simulink library "tip_assist_lib_support"  (Simulink 9.0)
settings: Solver=VariableStepAuto  StartTime=0.0  StopTime=10.0  RelTol=1e-3
undefined symbols (not defined in the file): g, timestep, TipAssistAdvEcmError_t, TipAssistCpmTipOffMode_t, TipAssistLiveWeighStatus_t, TipAssistPayloadType_t, TipAssistSecPfwStatus_t, TipAssistUnsecPfwStatus_t, toa_appNumber, toa_expectedBucketAngNoise, toa_imu_lpf_cutoff_hz, toa_imuBasicOrient, toa_liftBoreDia, toa_liftRodDia, toa_liveLpfCutoffHz, toa_liveSpillRateLpfCutoffHz, toa_mcGroundCombBucketAng, toa_mcGroundCombLiftNormAng, toa_mcGroundLiftNormAng, toa_noSlidingAngle, toa_payload_target_ov_val, toa_payloadTargetMin, toa_pfwLpfCutoffHz, toa_pfwResetLpfCutoffHz, toa_pfwResetStatsBound, toa_pfwResetStatsConf, toa_pfwTiltNormRackThresh, toa_pfwTravelExtentLower, toa_pfwTravelExtentUpper, toa_ratedPayload, toa_reposeMarginAng, toa_sendCpmLiveLpfCutoffHz, toa_sendToCpmMinPrecision, toa_tiltBoreDia, toa_tiltNumCyl, toa_tiltRodDia, toa_toolBcAngle, toa_toolBcLength
libraries: lib_CATutils_Utilities_ApplyName_v2 x113, simulink x18, tip_assist_lib x14, lib_CATutils_Filters_1Pole_LowPass x6, simulink_extras x5, lib_CATutils_Override x3, lib_CATutils_Hysteresis_Latch x3, lib_CATutils_Timer_Countdown x3, tip_assist_lib_support x2
(part 1 of 4)
settings Model: Creator=CurriSD  LastModifiedBy=CurriSD

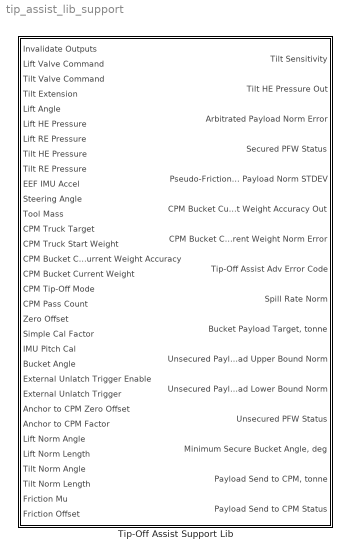
== system tip_assist_lib_support ==
  Tip-Off Assist Support Lib : Subsystem

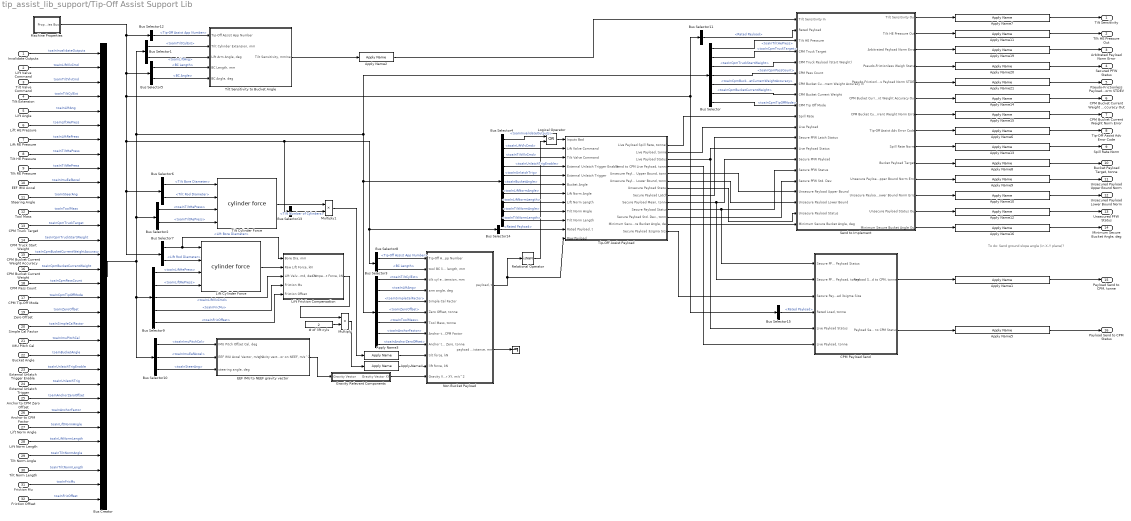
== system tip_assist_lib_support/Tip-Off Assist Support Lib ==
  note: To do: Send ground slope angle (in X-Y plane)?
  Invalidate Outputs : Inport
  Lift Valve Command : Inport  Port=2
  Tilt Valve Command : Inport  Port=3
  Tilt Extension : Inport  Port=4
  Lift Angle : Inport  Port=5
  Lift HE Pressure : Inport  Port=6
  Lift RE Pressure : Inport  Port=7
  Tilt HE Pressure : Inport  Port=8
  Tilt RE Pressure : Inport  Port=9
  EEF IMU Accel : Inport  Port=10
  Steering Angle : Inport  Port=11
  Tool Mass : Inport  Port=12
  CPM Truck Target : Inport  Port=13
  CPM Truck Start Weight : Inport  Port=14
  CPM Bucket Current Weight Accuracy : Inport  Port=15
  CPM Bucket Current Weight : Inport  Port=16
  CPM Tip-Off Mode : Inport  Port=17
  CPM Pass Count : Inport  Port=18
  Zero Offset : Inport  Port=19
  Simple Cal Factor : Inport  Port=20
  IMU Pitch Cal : Inport  Port=21
  Bucket Angle : Inport  Port=22
  External Unlatch Trigger Enable : Inport  Port=23
  External Unlatch Trigger : Inport  Port=24
  Anchor to CPM Zero Offset : Inport  Port=25
  Anchor to CPM Factor : Inport  Port=26
  Lift Norm Angle : Inport  Port=27
  Lift Norm Length : Inport  Port=28
  Tilt Norm Angle : Inport  Port=29
  Tilt Norm Length : Inport  Port=30
  Friction Mu : Inport  Port=31
  Friction Offset : Inport  Port=32
  " " : Terminator
  # of lift cyls : Constant  Value=2  OutDataTypeStr=single
  Apply Name1 : lib_CATutils_Utilities_ApplyName_v2/Apply Name  sigLabel='toa_outSendCpmPayload'  enTst=true
  Apply Name10 : lib_CATutils_Utilities_ApplyName_v2/Apply Name  sigLabel='toa_outUnsecPayloadNormLow'  enTst=true
  Apply Name11 : lib_CATutils_Utilities_ApplyName_v2/Apply Name  sigLabel='toa_outTiltHePress'  enTst=true
  Apply Name12 : lib_CATutils_Utilities_ApplyName_v2/Apply Name  sigLabel='toa_outUnsecPayloadStatus'  enTst=true
  Apply Name13 : lib_CATutils_Utilities_ApplyName_v2/Apply Name  sigLabel='toa_outSpillRateNorm'  enTst=true
  Apply Name14 : lib_CATutils_Utilities_ApplyName_v2/Apply Name  sigLabel='toa_outCpmAccu'  enTst=true
  Apply Name15 : lib_CATutils_Utilities_ApplyName_v2/Apply Name  sigLabel='toa_outCpmPayloadNormError'  enTst=true
  Apply Name16 : lib_CATutils_Utilities_ApplyName_v2/Apply Name  sigLabel='toa_outMinSecBucketAng'  enTst=true
  Apply Name19 : lib_CATutils_Utilities_ApplyName_v2/Apply Name  sigLabel='toa_outPayloadArbNormError'  enTst=true
  Apply Name2 : lib_CATutils_Utilities_ApplyName_v2/Apply Name  sigLabel='toa_tiltSensitivity'  enTst=true
  Apply Name20 : lib_CATutils_Utilities_ApplyName_v2/Apply Name  sigLabel='toa_outPfwStat'  enTst=true
  Apply Name21 : lib_CATutils_Utilities_ApplyName_v2/Apply Name  sigLabel='toa_outPfwPayloadNormStdev'  enTst=true
  Apply Name3 : lib_CATutils_Utilities_ApplyName_v2/Apply Name  sigLabel='toa_tiltForce'  enTst=true
  Apply Name4 : lib_CATutils_Utilities_ApplyName_v2/Apply Name  sigLabel='toa_liftForce'  enTst=true
  Apply Name5 : lib_CATutils_Utilities_ApplyName_v2/Apply Name  sigLabel='toa_outSendCpmStatus'  enTst=true
  Apply Name6 : lib_CATutils_Utilities_ApplyName_v2/Apply Name  sigLabel='toa_outAdvErrorCode'  enTst=true
  Apply Name7 : lib_CATutils_Utilities_ApplyName_v2/Apply Name  sigLabel='toa_outTiltSensToBucket'  enTst=true
  Apply Name8 : lib_CATutils_Utilities_ApplyName_v2/Apply Name  sigLabel='toa_outBucketPayloadTarget'  enTst=true
  Apply Name9 : lib_CATutils_Utilities_ApplyName_v2/Apply Name  sigLabel='toa_outUnsecPayloadNormUp'  enTst=true
  Bus Creator : BusCreator  Inputs=32
  Bus Selector : BusSelector  OutputSignals=toaInTiltHePress,toaInCpmTruckTarget,taoInCpmTruckStartWeight,toaInCpmPassCount,toaInCpmBucketCurrentWeightAccuracy,toaInCpmBucketCurrentWeight,toaInCpmTipOffMode
  Bus Selector1 : BusSelector  OutputSignals=toaInTiltCylExt,toaInLiftAng
  Bus Selector10 : BusSelector  OutputSignals=toaInImuPitchCal,toaInImuEefAccel,toaInSteerAng
  Bus Selector11 : BusSelector  OutputSignals=Rated Payload
  Bus Selector12 : BusSelector  OutputSignals=Tip-Off Assist App Number
  Bus Selector13 : BusSelector  OutputSignals=Tilt Number of Cylinders
  Bus Selector14 : BusSelector  OutputSignals=Rated Payload
  Bus Selector15 : BusSelector  OutputSignals=Rated Payload
  Bus Selector2 : BusSelector  OutputSignals=toaInTiltHePress,toaInTiltRePress
  Bus Selector3 : BusSelector  OutputSignals=toaInTiltCylExt,toaInLiftAng,toaInSimpleCalFactor,toaInZeroOffset,toaInToolMass,toaInAnchorFactor,toaInAnchorZeroOffset
  Bus Selector4 : BusSelector  OutputSignals=toaInInvalidateOutputs,toaInLiftVlvCmd,toaInTiltVlvCmd,toaInUnlatchTrigEnable,toaInUnlatchTrig,toaInBucketAngle,toaInLiftNormAngle,toaInLiftNormLength,toaInTiltNormAngle,toaInTiltNormLength
  Bus Selector5 : BusSelector  OutputSignals=BC Length,BC Angle
  Bus Selector6 : BusSelector  OutputSignals=Tilt Bore Diameter,Tilt Rod Diameter
  Bus Selector8 : BusSelector  OutputSignals=Tip-Off Assist App Number,BC Length
  Bus Selector9 : BusSelector  OutputSignals=toaInLiftHePress,toaInLiftRePress,toaInLiftVlvCmd,toaInFricMu,toaInFricOffset
  Bus Selector7 : BusSelector  OutputSignals=Lift Bore Diameter,Lift Rod Diameter
  CPM Payload Send : Subsystem
  EEF IMU to NEEF gravity vector : Subsystem
  Gravity Relevant Components : Subsystem
  Lift Cylinder Force : tip_assist_lib/cylinder force
  Lift Friction Compensation : Subsystem
  Logical Operator : Logic  Operator=OR  AllPortsSameDT=off  OutDataTypeStr=boolean
  Machine Properties : Subsystem
  Multiply : Product  SaturateOnIntegerOverflow=on  RndMeth=Zero  InputSameDT=on  OutDataTypeStr=Inherit: Same as first input
  Multiply1 : Product  SaturateOnIntegerOverflow=on  RndMeth=Zero  InputSameDT=on  OutDataTypeStr=Inherit: Same as first input
  Non Bucket Payload : Subsystem
  Relational Operator : RelationalOperator  Operator=isNaN  OutDataTypeStr=boolean  RndMeth=Simplest
  Send to Implement : Subsystem
  Tilt Cylinder Force : tip_assist_lib/cylinder force
  Tilt Sensitivity to Bucket Angle : Subsystem
  Tip-Off Assist Payload : Subsystem
  Tilt Sensitivity : Outport
  Tilt HE Pressure Out : Outport  Port=2
  Arbitrated Payload Norm Error : Outport  Port=3
  Secured PFW Status : Outport  Port=4
  Pseudo-Frictionless Payload Norm STDEV : Outport  Port=5
  CPM Bucket Current Weight Accuracy Out : Outport  Port=6
  CPM Bucket Current Weight Norm Error : Outport  Port=7
  Tip-Off Assist Adv Error Code : Outport  Port=8
  Spill Rate Norm : Outport  Port=9
  "Bucket Payload Target, tonne" : Outport  Port=10
  Unsecured Payload Upper Bound Norm : Outport  Port=11
  Unsecured Payload Lower Bound Norm : Outport  Port=12
  Unsecured PFW Status : Outport  Port=13
  "Minimum Secure Bucket Angle, deg" : Outport  Port=14
  "Payload Send to CPM, tonne" : Outport  Port=15
  Payload Send to CPM Status : Outport  Port=16
  wires:
  Apply Name4/1 -> Non Bucket Payload/11("lift force, kN")
  Apply Name3/1 -> Non Bucket Payload/10("tilt force, kN")
  Apply Name2/1 -> Send to Implement/1(Tilt Sensitivity In)
  Non Bucket Payload/2("payload distance, mm") -> " "/1
  Non Bucket Payload/1("payload, t") -> Relational Operator/1, Tip-Off Assist Payload/12(Raw Payload)
  Send to Implement/2(Tilt HE Pressure Out) -> Apply Name11/1
  Bus Selector/1 -> Send to Implement/3(Tilt HE Pressure)  "<toaInTiltHePress>"
  Bus Selector/6 -> Send to Implement/8(CPM Bucket Current Weight)  "<toaInCpmBucketCurrentWeight>"
  Bus Selector/5 -> Send to Implement/7(CPM Bucket Current Weight Accuracy In)  "<toaInCpmBucketCurrentWeightAccuracy>"
  Bus Selector/3 -> Send to Implement/5(CPM Truck Payload (Start Weight))  "<taoInCpmTruckStartWeight>"
  Bus Selector/7 -> Send to Implement/9(CPM Tip Off Mode)  "<toaInCpmTipOffMode>"
  Bus Selector/2 -> Send to Implement/4(CPM Truck Target)  "<toaInCpmTruckTarget>"
  Bus Selector3/5 -> Non Bucket Payload/7("Tool Mass, tonne")  "<toaInToolMass>"
  Tool Mass/1 -> Bus Creator/12  "toaInToolMass"
  Bus Selector10/3 -> EEF IMU to NEEF gravity vector/3("steering angle, deg")  "<toaInSteerAng>"
  Bus Selector10/2 -> EEF IMU to NEEF gravity vector/2("EEF IMU Accel Vector, m/s^2")  "<toaInImuEefAccel>"
  Bus Selector9/2 -> Lift Cylinder Force/4  "<toaInLiftRePress>"
  Bus Selector9/1 -> Lift Cylinder Force/3  "<toaInLiftHePress>"
  Bus Selector2/2 -> Tilt Cylinder Force/4  "<toaInTiltRePress>"
  Bus Selector2/1 -> Tilt Cylinder Force/3  "<toaInTiltHePress>"
  Lift Angle/1 -> Bus Creator/5  "toaInLiftAng"
  Tilt Extension/1 -> Bus Creator/4  "toaInTiltCylExt"
  Tilt Valve Command/1 -> Bus Creator/3  "toaInTiltVlvCmd"
  Lift Valve Command/1 -> Bus Creator/2  "toaInLiftVlvCmd"
  Lift RE Pressure/1 -> Bus Creator/7  "toaInLiftRePress"
  Bus Selector7/2 -> Lift Cylinder Force/2  "<Lift Rod Diameter>"
  Bus Selector4/3 -> Tip-Off Assist Payload/3(Tilt Valve Command)  "<toaInTiltVlvCmd>"
  Bus Selector4/2 -> Tip-Off Assist Payload/2(Lift Valve Command)  "<toaInLiftVlvCmd>"
  Tip-Off Assist Payload/1("Live Payload Spill Rate, tonne/s") -> Send to Implement/10(Spill Rate)
  Tip-Off Assist Payload/2("Live Payload, tonne") -> Send to Implement/11(Live Payload)
  Tip-Off Assist Payload/10(Secure Payload Status) -> CPM Payload Send/1(Secure PFW Payload Status), Send to Implement/15(Secure PFW Status)
  Bus Creator/1 -> Bus Selector1/1, Bus Selector3/1, Bus Selector4/1, Bus Selector/1, Bus Selector2/1, Bus Selector9/1, Bus Selector10/1
  Send to Implement/9(Spill Rate Norm) -> Apply Name13/1
  Send to Implement/8(Tip-Off Assist Adv Error Code) -> Apply Name6/1
  Send to Implement/4(Pseudo-Frictionless Weigh Status) -> Apply Name20/1
  Send to Implement/7(CPM Bucket Current Weight Norm Error) -> Apply Name15/1
  Send to Implement/6(CPM Bucket Current Weight Accuracy Out) -> Apply Name14/1
  Bus Selector8/2 -> Non Bucket Payload/2("tool BC link length, mm")  "<BC Length>"
  Bus Selector7/1 -> Lift Cylinder Force/1, Lift Friction Compensation/1("Bore Dia, mm")  "<Lift Bore Diameter>"
  Bus Selector6/2 -> Tilt Cylinder Force/2  "<Tilt Rod Diameter>"
  Bus Selector6/1 -> Tilt Cylinder Force/1  "<Tilt Bore Diameter>"
  Machine Properties/1(Properties Bus) -> Bus Selector12/1, Bus Selector11/1, Bus Selector15/1, Bus Selector7/1, Bus Selector6/1, Bus Selector8/1, Bus Selector14/1, Bus Selector13/1, Bus Selector5/1
  Bus Selector5/1 -> Tilt Sensitivity to Bucket Angle/4("BC Length, mm")  "<BC Length>"
  Bus Selector5/2 -> Tilt Sensitivity to Bucket Angle/5("BC Angle, deg")  "<BC Angle>"
  Gravity Relevant Components/1(Gravity Vector XY) -> Non Bucket Payload/12("Gravity Vector XY, m/s^2")
  EEF IMU to NEEF gravity vector/1("gravity vector on NEEF, m/s^2") -> Gravity Relevant Components/1(Gravity Vector)
  Bus Selector3/2 -> Non Bucket Payload/4("arm angle, deg")  "<toaInLiftAng>"
  Bus Selector3/1 -> Non Bucket Payload/3("tilt cyl extension, mm")  "<toaInTiltCylExt>"
  Bus Selector1/2 -> Tilt Sensitivity to Bucket Angle/3("Lift Arm Angle, deg")  "<toaInLiftAng>"
  Bus Selector1/1 -> Tilt Sensitivity to Bucket Angle/2("Tilt Cylinder Extension, mm")  "<toaInTiltCylExt>"
  Send to Implement/1(Tilt Sensitivity Out) -> Apply Name7/1
  Send to Implement/5(Pseudo-Frictionless Payload Norm STDEV) -> Apply Name21/1
  Send to Implement/3(Arbitrated Payload Norm Error) -> Apply Name19/1
  Tilt Sensitivity to Bucket Angle/1("Tilt Sensitivity, mm/rad") -> Apply Name2/1
  Steering Angle/1 -> Bus Creator/11  "toaInSteerAng"
  EEF IMU Accel/1 -> Bus Creator/10  "toaInImuEefAccel"
  # of lift cyls/1 -> Multiply/2
  Tilt Cylinder Force/1 -> Multiply1/1
  Multiply/1 -> Apply Name4/1
  Tilt RE Pressure/1 -> Bus Creator/9  "toaInTiltRePress"
  Lift HE Pressure/1 -> Bus Creator/6  "toaInLiftHePress"
  Tilt HE Pressure/1 -> Bus Creator/8  "toaInTiltHePress"
  Apply Name7/1 -> Tilt Sensitivity/1
  Apply Name11/1 -> Tilt HE Pressure Out/1
  Apply Name19/1 -> Arbitrated Payload Norm Error/1
  Apply Name20/1 -> Secured PFW Status/1
  Apply Name21/1 -> Pseudo-Frictionless Payload Norm STDEV/1
  Apply Name14/1 -> CPM Bucket Current Weight Accuracy Out/1
  Apply Name15/1 -> CPM Bucket Current Weight Norm Error/1
  Apply Name6/1 -> Tip-Off Assist Adv Error Code/1
  Apply Name13/1 -> Spill Rate Norm/1
  Bus Selector13/1 -> Multiply1/2  "<Tilt Number of Cylinders>"
  Multiply1/1 -> Apply Name3/1
  CPM Payload Send/1("Payload Send to CPM, tonne") -> Apply Name1/1
  CPM Payload Send/2(Payload Send to CPM Status) -> Apply Name5/1
  Invalidate Outputs/1 -> Bus Creator/1  "toaInInvalidateOutputs"
  CPM Truck Target/1 -> Bus Creator/13  "toaInCpmTruckTarget"
  CPM Truck Start Weight/1 -> Bus Creator/14  "taoInCpmTruckStartWeight"
  CPM Bucket Current Weight Accuracy/1 -> Bus Creator/15  "toaInCpmBucketCurrentWeightAccuracy"
  CPM Bucket Current Weight/1 -> Bus Creator/16  "toaInCpmBucketCurrentWeight"
  Bus Selector4/1 -> Logical Operator/1  "<toaInInvalidateOutputs>"
  Tip-Off Assist Payload/3(Live Payload Status) -> Send to Implement/13(Live Payload Status), CPM Payload Send/5(Live Payload Status)
  Bus Selector11/1 -> Send to Implement/2(Rated Payload)  "<Rated Payload>"
  Bus Selector8/1 -> Non Bucket Payload/1(Tip-Off Assist App Number)  "<Tip-Off Assist App Number>"
  Bus Selector12/1 -> Tilt Sensitivity to Bucket Angle/1(Tip-Off Assist App Number)  "<Tip-Off Assist App Number>"
  Bus Selector3/3 -> Non Bucket Payload/5(Simple Cal Factor)  "<toaInSimpleCalFactor>"
  Bus Selector3/4 -> Non Bucket Payload/6("Zero Offset, tonne")  "<toaInZeroOffset>"
  Bus Selector10/1 -> EEF IMU to NEEF gravity vector/1("IMU Pitch Offset Cal, deg")  "<toaInImuPitchCal>"
  Apply Name1/1 -> "Payload Send to CPM, tonne"/1
  Apply Name5/1 -> Payload Send to CPM Status/1
  Relational Operator/1 -> Logical Operator/2
  Logical Operator/1 -> Tip-Off Assist Payload/1(Inputs Bad)
  Bus Selector4/4 -> Tip-Off Assist Payload/4(External Unlatch Trigger Enable)  "<toaInUnlatchTrigEnable>"
  Bus Selector4/5 -> Tip-Off Assist Payload/5(External Unlatch Trigger)  "<toaInUnlatchTrig>"
  Bus Selector4/6 -> Tip-Off Assist Payload/6(Bucket Angle)  "<toaInBucketAngle>"
  Send to Implement/10(Bucket Payload Target) -> Apply Name8/1
  Apply Name8/1 -> "Bucket Payload Target, tonne"/1
  Tip-Off Assist Payload/9("Secure Payload Mean, tonne") -> Send to Implement/14(Secure PFW Payload), CPM Payload Send/2("Secure PFW Payload, tonne")
  Tip-Off Assist Payload/11("Secure Payload Std. Dev., tonne") -> Send to Implement/16(Secure PFW Std. Dev.)
  Bus Selector3/6 -> Non Bucket Payload/8(Anchor to CPM Factor)  "<toaInAnchorFactor>"
  Bus Selector3/7 -> Non Bucket Payload/9("Anchor to CPM Zero, tonne")  "<toaInAnchorZeroOffset>"
  Bus Selector14/1 -> Tip-Off Assist Payload/11("Rated Payload, t")  "<Rated Payload>"
  Tip-Off Assist Payload/13(Secure Payload 3sigma Size) -> CPM Payload Send/3(Secure Payload 3sigma Size)
  Bus Selector15/1 -> CPM Payload Send/4("Rated Load, tonne")  "<Rated Payload>"
  Tip-Off Assist Payload/8(Secure Payload Latch) -> Send to Implement/12(Secure PFW Latch Status)
  Tip-Off Assist Payload/5("Unsecure Payload Upper Bound, tonne") -> Send to Implement/17(Unsecure Payload Upper Bound)
  Tip-Off Assist Payload/6("Unsecure Payload Lower Bound, tonne") -> Send to Implement/18(Unsecure Payload Lower Bound)
  Tip-Off Assist Payload/7(Unsecure Payload Status) -> Send to Implement/19(Unsecure Payload Status)
  Send to Implement/11(Unsecure Payload Upper Bound Norm Error) -> Apply Name9/1
  Send to Implement/12(Unsecure Payload Lower Bound Norm Error) -> Apply Name10/1
  Send to Implement/13(Unsecure Payload Status Out) -> Apply Name12/1
  Apply Name9/1 -> Unsecured Payload Upper Bound Norm/1
  Apply Name10/1 -> Unsecured Payload Lower Bound Norm/1
  Apply Name12/1 -> Unsecured PFW Status/1
  Tip-Off Assist Payload/12("Minimum Secure Bucket Angle, deg") -> Send to Implement/20("Minimum Secure Bucket Angle, deg")
  Send to Implement/14(Minimum Secure Bucket Angle Out) -> Apply Name16/1
  Apply Name16/1 -> "Minimum Secure Bucket Angle, deg"/1
  Tilt Norm Angle/1 -> Bus Creator/29  "toaInTiltNormAngle"
  Tilt Norm Length/1 -> Bus Creator/30  "toaInTiltNormLength"
  Bus Selector4/7 -> Tip-Off Assist Payload/7(Lift Norm Angle)  "<toaInLiftNormAngle>"
  Bus Selector4/8 -> Tip-Off Assist Payload/8(Lift Norm Length)  "<toaInLiftNormLength>"
  Bus Selector4/9 -> Tip-Off Assist Payload/9(Tilt Norm Angle)  "<toaInTiltNormAngle>"
  Bus Selector4/10 -> Tip-Off Assist Payload/10(Tilt Norm Length)  "<toaInTiltNormLength>"
  CPM Pass Count/1 -> Bus Creator/17  "toaInCpmPassCount"
  CPM Tip-Off Mode/1 -> Bus Creator/18  "toaInCpmTipOffMode"
  Zero Offset/1 -> Bus Creator/19  "toaInZeroOffset"
  Simple Cal Factor/1 -> Bus Creator/20  "toaInSimpleCalFactor"
  IMU Pitch Cal/1 -> Bus Creator/21  "toaInImuPitchCal"
  Bucket Angle/1 -> Bus Creator/22  "toaInBucketAngle"
  External Unlatch Trigger Enable/1 -> Bus Creator/23  "toaInUnlatchTrigEnable"
  External Unlatch Trigger/1 -> Bus Creator/24  "toaInUnlatchTrig"
  Anchor to CPM Zero Offset/1 -> Bus Creator/25  "toaInAnchorZeroOffset"
  Anchor to CPM Factor/1 -> Bus Creator/26  "toaInAnchorFactor"
  Lift Norm Angle/1 -> Bus Creator/27  "toaInLiftNormAngle"
  Lift Norm Length/1 -> Bus Creator/28  "toaInLiftNormLength"
  Bus Selector/4 -> Send to Implement/6(CPM Pass Count)  "<toaInCpmPassCount>"
  Tip-Off Assist Payload/4("Send to CPM Live Payload, tonne") -> CPM Payload Send/6("Live Payload, tonne")
  Lift Cylinder Force/1 -> Lift Friction Compensation/2("Raw Lift Force, kN")
  Bus Selector9/3 -> Lift Friction Compensation/3("Lift Valve Cmd, dec %")  "<toaInLiftVlvCmd>"
  Lift Friction Compensation/1("Compensated Lift Force, kN") -> Multiply/1
  Friction Mu/1 -> Bus Creator/31  "toaInFricMu"
  Friction Offset/1 -> Bus Creator/32  "toaInFricOffset"
  Bus Selector9/5 -> Lift Friction Compensation/5(Friction Offset)  "<toaInFricOffset>"
  Bus Selector9/4 -> Lift Friction Compensation/4(Friction Mu)  "<toaInFricMu>"

== system tip_assist_lib_support/Tip-Off Assist Support Lib/CPM Payload Send ==
  Secure PFW Payload Status : Inport
  "Secure PFW Payload, tonne" : Inport  Port=2
  Secure Payload 3sigma Size : Inport  Port=3
  "Rated Load, tonne" : Inport  Port=4
  Live Payload Status : Inport  Port=5
  "Live Payload, tonne" : Inport  Port=6
  Apply Name1 : lib_CATutils_Utilities_ApplyName_v2/Apply Name  sigLabel='toa_sendCpmPfwIsPrecise'  enTst=true
  Apply Name9 : lib_CATutils_Utilities_ApplyName_v2/Apply Name  sigLabel='toa_sendCpmPfwSecSize'  enTst=true
  Constant : Constant  Value=toa_sendToCpmMinPrecision
  Divide : Product  Inputs=*/
  MATLAB Function : MATLAB Function  TreatAsAtomicUnit=on
  Relational Operator : RelationalOperator  Operator=<=  OutDataTypeStr=boolean  RndMeth=Simplest
  "Payload Send to CPM, tonne" : Outport
  Payload Send to CPM Status : Outport  Port=2
  wires:
  Secure PFW Payload Status/1 -> MATLAB Function/1(pfwStatus)
  "Secure PFW Payload, tonne"/1 -> MATLAB Function/2(pfwPayload)
  "Live Payload, tonne"/1 -> MATLAB Function/5(livePayload)
  Live Payload Status/1 -> MATLAB Function/4(liveStatus)
  MATLAB Function/1(outPayload) -> "Payload Send to CPM, tonne"/1
  MATLAB Function/2(outStatus) -> Payload Send to CPM Status/1
  Secure Payload 3sigma Size/1 -> Apply Name9/1
  Divide/1 -> Relational Operator/1
  "Rated Load, tonne"/1 -> Divide/2
  Relational Operator/1 -> Apply Name1/1
  Constant/1 -> Relational Operator/2
  Apply Name9/1 -> Divide/1
  Apply Name1/1 -> MATLAB Function/3(pfwIsPrecise)

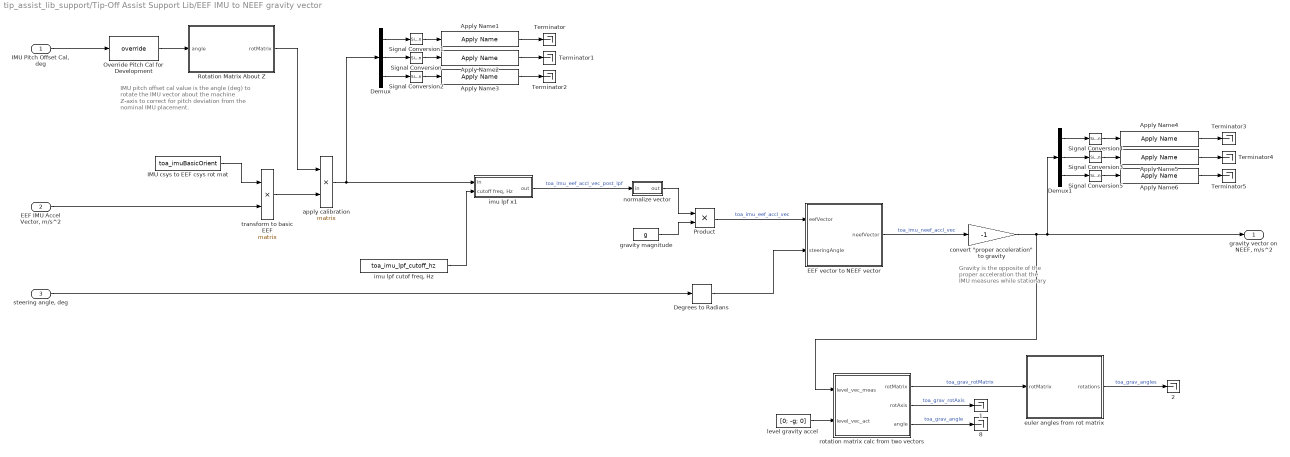
== system tip_assist_lib_support/Tip-Off Assist Support Lib/EEF IMU to NEEF gravity vector ==
  note: IMU pitch offset cal value is the angle (deg) to rotate the IMU vector about the machine Z-axis to correct for pitch deviation from the nominal IMU placement.
  note: Gravity is the opposite of the proper acceleration that the IMU measures while stationary
  "IMU Pitch Offset Cal, deg" : Inport
  "EEF IMU Accel Vector, m/s^2" : Inport  Port=2
  "steering angle, deg" : Inport  Port=3
  " 1" : Terminator
  " 2" : Terminator
  " 8" : Terminator
  Apply Name1 : lib_CATutils_Utilities_ApplyName_v2/Apply Name  sigLabel='toa_imuRawEefAcclX'  enTst=true
  Apply Name2 : lib_CATutils_Utilities_ApplyName_v2/Apply Name  sigLabel='toa_imuRawEefAcclY'  enTst=true
  Apply Name3 : lib_CATutils_Utilities_ApplyName_v2/Apply Name  sigLabel='toa_imuRawEefAcclZ'  enTst=true
  Apply Name4 : lib_CATutils_Utilities_ApplyName_v2/Apply Name  sigLabel='toa_imuNeefGravX'  enTst=true
  Apply Name5 : lib_CATutils_Utilities_ApplyName_v2/Apply Name  sigLabel='toa_imuNeefGravY'  enTst=true
  Apply Name6 : lib_CATutils_Utilities_ApplyName_v2/Apply Name  sigLabel='toa_imuNeefGravZ'  enTst=true
  Degrees to Radians : simulink_extras/Transformations/Degrees to Radians
  Demux : Demux  Outputs=3
  Demux1 : Demux  Outputs=3
  EEF vector to NEEF vector : MATLAB Function  TreatAsAtomicUnit=on
  IMU csys to EEF csys rot mat : Constant  Value=toa_imuBasicOrient  VectorParams1D=off  OutDataTypeStr=single  SampleTime=-1
  Override Pitch Cal for Development : lib_CATutils_Override/override  ovType=OV if OV ~= Pass  extOV=off  ov_value=toa_imuCalPitchAngOv  extPass=off  pass_value=360  extRange=off  ov_max=100  ov_min=1  extCond=off  ov_cond=toa_imuCalPitchAngOv  extTF=off  ov_TrueComp=1  ov_FalseComp=2
  Product : Product  Inputs=**  OutDataTypeStr=Inherit: Same as first input
  Rotation Matrix About Z : MATLAB Function  TreatAsAtomicUnit=on
  Signal Conversion{,1..5} (6 alike) : SignalConversion  OverrideOpt=on
  Terminator{,1..5} (6 alike) : Terminator
  apply calibration : Product  Multiplication=Matrix(*)  SaturateOnIntegerOverflow=on  RndMeth=Zero  OutDataTypeStr=Inherit: Same as first input
  "convert \"proper acceleration\" to gravity" : Gain  Gain=-1  SaturateOnIntegerOverflow=on  OutDataTypeStr=Inherit: Same as input  ParamDataTypeStr=Inherit: Same as input
  euler angles from rot matrix : MATLAB Function  TreatAsAtomicUnit=on
  gravity magnitude : Constant  Value=g  OutDataTypeStr=single  SampleTime=timestep
  "imu lpf cutof freq, Hz" : Constant  Value=toa_imu_lpf_cutoff_hz  OutDataTypeStr=single  SampleTime=timestep
  imu lpf x1 : Subsystem
  level gravity accel : Constant  Value=[0; -g; 0]  OutDataTypeStr=single  SampleTime=-1
  normalize vector : Subsystem
  rotation matrix calc from two vectors : MATLAB Function  TreatAsAtomicUnit=on
  transform to basic EEF : Product  Multiplication=Matrix(*)  SaturateOnIntegerOverflow=on  RndMeth=Zero  OutDataTypeStr=Inherit: Same as first input
  "gravity vector on NEEF, m/s^2" : Outport
  wires:
  level gravity accel/1 -> rotation matrix calc from two vectors/2(level_vec_act)
  rotation matrix calc from two vectors/3(angle) -> " 8"/1  "toa_grav_angle"
  rotation matrix calc from two vectors/2(rotAxis) -> " 1"/1  "toa_grav_rotAxis"
  rotation matrix calc from two vectors/1(rotMatrix) -> euler angles from rot matrix/1(rotMatrix)  "toa_grav_rotMatrix"
  "EEF IMU Accel Vector, m/s^2"/1 -> transform to basic EEF/2
  "convert \"proper acceleration\" to gravity"/1 -> Demux1/1, "gravity vector on NEEF, m/s^2"/1, rotation matrix calc from two vectors/1(level_vec_meas)
  IMU csys to EEF csys rot mat/1 -> transform to basic EEF/1
  transform to basic EEF/1 -> apply calibration/2
  Rotation Matrix About Z/1(rotMatrix) -> apply calibration/1
  Override Pitch Cal for Development/1 -> Rotation Matrix About Z/1(angle)
  gravity magnitude/1 -> Product/2
  imu lpf x1/1(out) -> normalize vector/1(in)  "toa_imu_eef_accl_vec_post_lpf"
  normalize vector/1(out) -> Product/1
  EEF vector to NEEF vector/1(neefVector) -> "convert \"proper acceleration\" to gravity"/1  "toa_imu_neef_accl_vec"
  "steering angle, deg"/1 -> Degrees to Radians/1
  Product/1 -> EEF vector to NEEF vector/1(eefVector)  "toa_imu_eef_accl_vec"
  Degrees to Radians/1 -> EEF vector to NEEF vector/2(steeringAngle)
  "imu lpf cutof freq, Hz"/1 -> imu lpf x1/2("cutoff freq, Hz")
  euler angles from rot matrix/1(rotations) -> " 2"/1  "toa_grav_angles"
  "IMU Pitch Offset Cal, deg"/1 -> Override Pitch Cal for Development/1
  apply calibration/1 -> Demux/1, imu lpf x1/1(in)
  Demux/2 -> Signal Conversion/1
  Demux/1 -> Signal Conversion1/1
  Signal Conversion1/1 -> Apply Name1/1
  Apply Name1/1 -> Terminator/1
  Signal Conversion/1 -> Apply Name2/1
  Signal Conversion2/1 -> Apply Name3/1
  Demux/3 -> Signal Conversion2/1
  Apply Name2/1 -> Terminator1/1
  Apply Name3/1 -> Terminator2/1
  Apply Name6/1 -> Terminator5/1
  Apply Name5/1 -> Terminator4/1
  Demux1/3 -> Signal Conversion5/1
  Signal Conversion5/1 -> Apply Name6/1
  Signal Conversion3/1 -> Apply Name5/1
  Apply Name4/1 -> Terminator3/1
  Signal Conversion4/1 -> Apply Name4/1
  Demux1/1 -> Signal Conversion4/1
  Demux1/2 -> Signal Conversion3/1

== system tip_assist_lib_support/Tip-Off Assist Support Lib/Gravity Relevant Components ==
  Gravity Vector : Inport
  " neef gravity vector z" : Terminator
  " neef gravity vector z1" : Terminator
  " neef gravity vector z2" : Terminator
  Add : Sum
  Apply Name3 : lib_CATutils_Utilities_ApplyName_v2/Apply Name  sigLabel='toa_imuNeefPitch'  enTst=true
  Constant : Constant  Value=90  SampleTime=-1
  Demux : Demux  Outputs=3
  Magnitude : Subsystem
  Override : lib_CATutils_Override/override  ovType=OV if OV ~= Pass  extOV=off  ov_value=toa_grav_y_ov_val  extPass=off  pass_value=0  extRange=off  ov_max=100  ov_min=1  extCond=off  ov_cond=0  extTF=off  ov_TrueComp=1  ov_FalseComp=2
  Override1 : lib_CATutils_Override/override  ovType=OV if OV ~= Pass  extOV=off  ov_value=toa_grav_x_ov_val  extPass=off  pass_value=0  extRange=off  ov_max=100  ov_min=1  extCond=off  ov_cond=0  extTF=off  ov_TrueComp=1  ov_FalseComp=2
  Radians to Degrees : simulink_extras/Transformations/Radians to Degrees
  Trigonometric Function : Trigonometry  Operator=atan2  OutputSignalType=real
  Vector Concatenate1 : Concatenate  Mode=Multidimensional array
  "convert \"proper acceleration\" to gravity1" : Gain  Gain=-1  SaturateOnIntegerOverflow=on  OutDataTypeStr=Inherit: Same as input  ParamDataTypeStr=Inherit: Same as input
  Gravity Vector XY : Outport
  wires:
  Vector Concatenate1/1 -> Gravity Vector XY/1, Magnitude/1(vector)
  Demux/1 -> Override1/1
  Demux/2 -> Override/1
  Demux/3 -> " neef gravity vector z"/1
  Override/1 -> Trigonometric Function/1, Vector Concatenate1/2
  Trigonometric Function/1 -> Radians to Degrees/1
  Magnitude/1(magnitude) -> " neef gravity vector z2"/1  "toa_grav_neef_xy_mag"
  Override1/1 -> Vector Concatenate1/1, Trigonometric Function/2
  Gravity Vector/1 -> Demux/1
  Radians to Degrees/1 -> Add/1
  Constant/1 -> Add/2
  Add/1 -> "convert \"proper acceleration\" to gravity1"/1
  "convert \"proper acceleration\" to gravity1"/1 -> Apply Name3/1
  Apply Name3/1 -> " neef gravity vector z1"/1

== system tip_assist_lib_support/Tip-Off Assist Support Lib/Lift Friction Compensation ==
  "Bore Dia, mm" : Inport
  "Raw Lift Force, kN" : Inport  Port=2
  "Lift Valve Cmd, dec %" : Inport  Port=3
  Friction Mu : Inport  Port=4
  Friction Offset : Inport  Port=5
  Apply Name : lib_CATutils_Utilities_ApplyName_v2/Apply Name  sigLabel='toa_fcLiftForceComp'  enTst=true
  Apply Name1 : lib_CATutils_Utilities_ApplyName_v2/Apply Name  sigLabel='toa_fcLiftForceRaw'  enTst=true
  Divide : Product  Inputs=/*
  MATLAB Function : MATLAB Function  TreatAsAtomicUnit=on
  Product : Product
  diameter to area : tip_assist_lib/cylinder force/diameter to area
  kN per mm^2 to kPa : Gain  Gain=1e6
  kPa to kN per mm^2 : Gain  Gain=1e-6
  "Compensated Lift Force, kN" : Outport
  wires:
  "Raw Lift Force, kN"/1 -> Apply Name1/1
  "Lift Valve Cmd, dec %"/1 -> MATLAB Function/2(liftCmd)
  Friction Offset/1 -> MATLAB Function/4(fricOffset)
  Friction Mu/1 -> MATLAB Function/3(fricCoeff)
  MATLAB Function/1(compPress) -> kPa to kN per mm^2/1
  Apply Name/1 -> "Compensated Lift Force, kN"/1
  Apply Name1/1 -> Divide/2
  "Bore Dia, mm"/1 -> diameter to area/1
  Divide/1 -> kN per mm^2 to kPa/1
  Product/1 -> Apply Name/1
  diameter to area/1 -> Divide/1, Product/1
  kN per mm^2 to kPa/1 -> MATLAB Function/1(rawPress)
  kPa to kN per mm^2/1 -> Product/2

== system tip_assist_lib_support/Tip-Off Assist Support Lib/Machine Properties ==
  # of tilt cyls : Constant  Value=toa_tiltNumCyl  OutDataTypeStr=single  SampleTime=-1
  "BC Angle, deg" : Constant  Value=toa_toolBcAngle  OutDataTypeStr=single
  Bus Creator : BusCreator  Inputs=9
  "Length btw BC pins, mm" : Constant  Value=toa_toolBcLength  OutDataTypeStr=single  SampleTime=-1
  "Rated Payload, tonne" : Constant  Value=toa_ratedPayload  OutDataTypeStr=single  SampleTime=-1
  Tip-Off Assist App Number : Constant  Value=toa_appNumber  OutDataTypeStr=uint32  SampleTime=-1
  "lift bore dia, mm" : Constant  Value=toa_liftBoreDia  OutDataTypeStr=single
  "lift rod dia, mm" : Constant  Value=toa_liftRodDia  OutDataTypeStr=single
  "tilt bore dia, mm" : Constant  Value=toa_tiltBoreDia  OutDataTypeStr=single
  "tilt rod dia, mm" : Constant  Value=toa_tiltRodDia  OutDataTypeStr=single
  Properties Bus : Outport
  wires:
  "lift rod dia, mm"/1 -> Bus Creator/5  "Lift Rod Diameter"
  Bus Creator/1 -> Properties Bus/1
  "tilt rod dia, mm"/1 -> Bus Creator/3  "Tilt Rod Diameter"
  "lift bore dia, mm"/1 -> Bus Creator/4  "Lift Bore Diameter"
  "tilt bore dia, mm"/1 -> Bus Creator/2  "Tilt Bore Diameter"
  "Length btw BC pins, mm"/1 -> Bus Creator/7  "BC Length"
  "BC Angle, deg"/1 -> Bus Creator/6  "BC Angle"
  "Rated Payload, tonne"/1 -> Bus Creator/8  "Rated Payload"
  Tip-Off Assist App Number/1 -> Bus Creator/1  "Tip-Off Assist App Number"
  # of tilt cyls/1 -> Bus Creator/9  "Tilt Number of Cylinders"

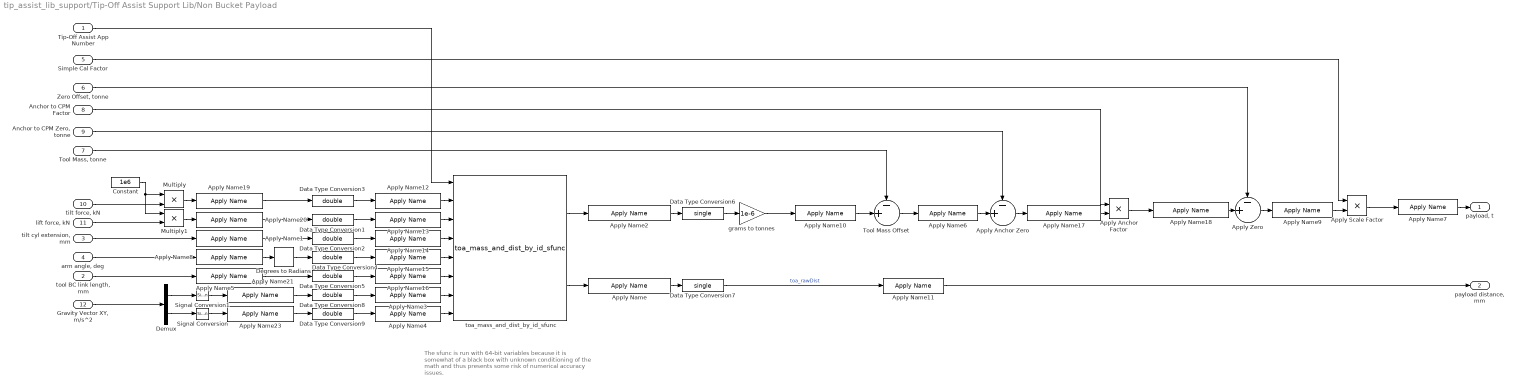
== system tip_assist_lib_support/Tip-Off Assist Support Lib/Non Bucket Payload ==
  note: The sfunc is run with 64-bit variables because it is somewhat of a black box with unknown conditioning of the math and thus presents some risk of numerical accuracy issues.
  Tip-Off Assist App Number : Inport
  "tool BC link length, mm" : Inport  Port=2
  "tilt cyl extension, mm" : Inport  Port=3
  "arm angle, deg" : Inport  Port=4
  Simple Cal Factor : Inport  Port=5
  "Zero Offset, tonne" : Inport  Port=6
  "Tool Mass, tonne" : Inport  Port=7
  Anchor to CPM Factor : Inport  Port=8
  "Anchor to CPM Zero, tonne" : Inport  Port=9
  "tilt force, kN" : Inport  Port=10
  "lift force, kN" : Inport  Port=11
  "Gravity Vector XY, m/s^2" : Inport  Port=12
  Apply Anchor Factor : Product
  Apply Anchor Zero : Sum  Inputs=-+|  SaturateOnIntegerOverflow=on  InputSameDT=on  OutDataTypeStr=Inherit: Same as first input
  Apply Name : lib_CATutils_Utilities_ApplyName_v2/Apply Name  sigLabel='toa_sfuncOutRawDist'  enTst=true
  Apply Name1 : lib_CATutils_Utilities_ApplyName_v2/Apply Name  sigLabel='toa_sfuncInTiltExt'  enTst=true
  Apply Name10 : lib_CATutils_Utilities_ApplyName_v2/Apply Name  sigLabel='toa_sfuncOutRawMassTonne'  enTst=true
  Apply Name11 : lib_CATutils_Utilities_ApplyName_v2/Apply Name  sigLabel='toa_rawDist'  enTst=true
  Apply Name12 : lib_CATutils_Utilities_ApplyName_v2/Apply Name  sigLabel='toa_sfuncInRawTiltForce'  enTst=true
  Apply Name13 : lib_CATutils_Utilities_ApplyName_v2/Apply Name  sigLabel='toa_sfuncInRawLiftForce'  enTst=true
  Apply Name14 : lib_CATutils_Utilities_ApplyName_v2/Apply Name  sigLabel='toa_sfuncInRawTiltExt'  enTst=true
  Apply Name15 : lib_CATutils_Utilities_ApplyName_v2/Apply Name  sigLabel='toa_sfuncInRawLiftAng'  enTst=true
  Apply Name16 : lib_CATutils_Utilities_ApplyName_v2/Apply Name  sigLabel='toa_sfuncInRawBcLength'  enTst=true
  Apply Name17 : lib_CATutils_Utilities_ApplyName_v2/Apply Name  sigLabel='toa_payloadAncZeroed'  enTst=true
  Apply Name18 : lib_CATutils_Utilities_ApplyName_v2/Apply Name  sigLabel='toa_payloadAncAdjusted'  enTst=true
  Apply Name19 : lib_CATutils_Utilities_ApplyName_v2/Apply Name  sigLabel='toa_sfuncInTiltForce'  enTst=true
  Apply Name2 : lib_CATutils_Utilities_ApplyName_v2/Apply Name  sigLabel='toa_sfuncOutRawMass'  enTst=true
  Apply Name20 : lib_CATutils_Utilities_ApplyName_v2/Apply Name  sigLabel='toa_sfuncInLiftForce'  enTst=true
  Apply Name21 : lib_CATutils_Utilities_ApplyName_v2/Apply Name  sigLabel='toa_sfuncInGravX'  enTst=true
  Apply Name23 : lib_CATutils_Utilities_ApplyName_v2/Apply Name  sigLabel='toa_sfuncInGravY'  enTst=true
  Apply Name3 : lib_CATutils_Utilities_ApplyName_v2/Apply Name  sigLabel='toa_sfuncInRawGravX'  enTst=true
  Apply Name4 : lib_CATutils_Utilities_ApplyName_v2/Apply Name  sigLabel='toa_sfuncInRawGravY'  enTst=true
  Apply Name5 : lib_CATutils_Utilities_ApplyName_v2/Apply Name  sigLabel='toa_sfuncInBcLength'  enTst=true
  Apply Name6 : lib_CATutils_Utilities_ApplyName_v2/Apply Name  sigLabel='toa_rawPayload'  enTst=true
  Apply Name7 : lib_CATutils_Utilities_ApplyName_v2/Apply Name  sigLabel='toa_payloadAdjusted'  enTst=true
  Apply Name8 : lib_CATutils_Utilities_ApplyName_v2/Apply Name  sigLabel='toa_sfuncInLiftAng'  enTst=true
  Apply Name9 : lib_CATutils_Utilities_ApplyName_v2/Apply Name  sigLabel='toa_payloadZeroed'  enTst=true
  Apply Scale Factor : Product
  Apply Zero : Sum  Inputs=-+|  SaturateOnIntegerOverflow=on  InputSameDT=on  OutDataTypeStr=Inherit: Same as first input
  Constant : Constant  Value=1e6  OutDataTypeStr=single
  Data Type Conversion{1..5,8..9} (7 alike) : DataTypeConversion  OutDataTypeStr=double  SaturateOnIntegerOverflow=on  RndMeth=Zero
      settings: AttributesFormatString=Output Data Type: %<OutDataTypeStr>\n
  Data Type Conversion6 : DataTypeConversion  OutDataTypeStr=single  SaturateOnIntegerOverflow=on  RndMeth=Zero
      settings: AttributesFormatString=Output Data Type: %<OutDataTypeStr>\n
  Data Type Conversion7 : DataTypeConversion  OutDataTypeStr=single  SaturateOnIntegerOverflow=on  RndMeth=Zero
      settings: AttributesFormatString=Output Data Type: %<OutDataTypeStr>\n
  Degrees to Radians : simulink_extras/Transformations/Degrees to Radians
  Demux : Demux  Outputs=2
  Multiply : Product  SaturateOnIntegerOverflow=on  RndMeth=Zero  InputSameDT=on  OutDataTypeStr=Inherit: Same as first input
  Multiply1 : Product  SaturateOnIntegerOverflow=on  RndMeth=Zero  InputSameDT=on  OutDataTypeStr=Inherit: Same as first input
  Signal Conversion : SignalConversion  OverrideOpt=on
  Signal Conversion1 : SignalConversion  OverrideOpt=on
  Tool Mass Offset : Sum  Inputs=-+|  SaturateOnIntegerOverflow=on  InputSameDT=on  OutDataTypeStr=Inherit: Same as first input
  grams to tonnes : Gain  Gain=1e-6  SaturateOnIntegerOverflow=on  OutDataTypeStr=Inherit: Same as input  ParamDataTypeStr=Inherit: Same as input
  toa_mass_and_dist_by_id_sfunc : S-Function  FunctionName=toa_mass_and_dist_by_id_sfunc  SFunctionDeploymentMode=off  EnableBusSupport=off  mask(Legacy Function){SFunctionSpec=void toa_mass_and_dist_by_id(uint32 u1, double u2, double u3, double u4, double u5, double u6, double u7, double u8, double y1[1], double y2[1]), ShowSpec=off}
      mask prompts: ShowSpec "Display function specification"
      mask help:
      | This block allows you to call the legacy functions specified by the following Legacy Code Tool definition:
      | def.SFunctionName = 'toa_mass_and_dist_by_id_sfunc';
      | def.OutputFcnSpec = 'void toa_mass_and_dist_by_id(uint32 u1, double u2, double u3, double u4, double u5, double u6, double u7, double u8, double y1[1], double y2[1])';
      | def.HeaderFiles = {'tipoff_assist.h'};
      | def.SourceFiles = {'tipoff_assist.c'};
      | def.IncPaths = {'./c_src'};
      mask Help: <p>This block was generated automatically by the Legacy Code Tool. For detailed help on this tool, call<a href="matlab:legacy_code('help')"> legacy_code('help')</a>.</p>
      mask Callback ShowSpec:
      | if strcmp(get_param(gcbh, 'ShowSpec'), 'on')
      |   set_param(gcbh, 'MaskDisplay', sprintf('fprintf(''%s'');', get_param(gcbh, 'SFunctionSpec')));
      | else
      |   set_param(gcbh, 'MaskDisplay', sprintf('fprintf(''%s'');', get_param(gcbh, 'FunctionName')));
      | end
      mask Display: fprintf('%s','void toa_mass_and_dist_by_id(uint32 u1, double u2, double u3, double u4, double u5, double u6, double u7, double u8, double y1[1], double y2[1])');
  "payload, t" : Outport
  "payload distance, mm" : Outport  Port=2
  wires:
  "arm angle, deg"/1 -> Apply Name8/1
  Degrees to Radians/1 -> Data Type Conversion4/1
  Apply Name8/1 -> Degrees to Radians/1
  Multiply/1 -> Apply Name19/1
  Multiply1/1 -> Apply Name20/1
  "tilt cyl extension, mm"/1 -> Apply Name1/1
  Demux/1 -> Signal Conversion1/1
  Demux/2 -> Signal Conversion/1
  Apply Name5/1 -> Data Type Conversion5/1
  Apply Name2/1 -> Data Type Conversion6/1
  Apply Name/1 -> Data Type Conversion7/1
  grams to tonnes/1 -> Apply Name10/1
  "Gravity Vector XY, m/s^2"/1 -> Demux/1
  "Tool Mass, tonne"/1 -> Tool Mass Offset/1
  Data Type Conversion9/1 -> Apply Name4/1
  Data Type Conversion8/1 -> Apply Name3/1
  Data Type Conversion7/1 -> Apply Name11/1  "toa_rawDist"
  Data Type Conversion6/1 -> grams to tonnes/1
  Data Type Conversion5/1 -> Apply Name16/1
  Data Type Conversion4/1 -> Apply Name15/1
  Data Type Conversion2/1 -> Apply Name14/1
  Data Type Conversion1/1 -> Apply Name13/1
  Data Type Conversion3/1 -> Apply Name12/1
  Constant/1 -> Multiply/1, Multiply1/1
  "tool BC link length, mm"/1 -> Apply Name5/1
  "lift force, kN"/1 -> Multiply1/2
  "tilt force, kN"/1 -> Multiply/2
  toa_mass_and_dist_by_id_sfunc/2 -> Apply Name/1
  toa_mass_and_dist_by_id_sfunc/1 -> Apply Name2/1
  Tip-Off Assist App Number/1 -> toa_mass_and_dist_by_id_sfunc/1
  Apply Name4/1 -> toa_mass_and_dist_by_id_sfunc/8
  Apply Name3/1 -> toa_mass_and_dist_by_id_sfunc/7
  Apply Name16/1 -> toa_mass_and_dist_by_id_sfunc/6
  Apply Name15/1 -> toa_mass_and_dist_by_id_sfunc/5
  Apply Name14/1 -> toa_mass_and_dist_by_id_sfunc/4
  Apply Name13/1 -> toa_mass_and_dist_by_id_sfunc/3
  Apply Name12/1 -> toa_mass_and_dist_by_id_sfunc/2
  Tool Mass Offset/1 -> Apply Name6/1
  "Zero Offset, tonne"/1 -> Apply Zero/1
  Simple Cal Factor/1 -> Apply Scale Factor/1
  Apply Zero/1 -> Apply Name9/1
  Apply Scale Factor/1 -> Apply Name7/1
  Apply Name1/1 -> Data Type Conversion2/1
  Signal Conversion/1 -> Apply Name23/1
  Signal Conversion1/1 -> Apply Name21/1
  Apply Name6/1 -> Apply Anchor Zero/2
  Apply Name7/1 -> "payload, t"/1
  Apply Name9/1 -> Apply Scale Factor/2
  Apply Name10/1 -> Tool Mass Offset/2
  Apply Name11/1 -> "payload distance, mm"/1
  Apply Anchor Zero/1 -> Apply Name17/1
  Apply Name17/1 -> Apply Anchor Factor/2
  Apply Anchor Factor/1 -> Apply Name18/1
  Apply Name18/1 -> Apply Zero/2
  Anchor to CPM Factor/1 -> Apply Anchor Factor/1
  "Anchor to CPM Zero, tonne"/1 -> Apply Anchor Zero/1
  Apply Name19/1 -> Data Type Conversion3/1
  Apply Name20/1 -> Data Type Conversion1/1
  Apply Name21/1 -> Data Type Conversion8/1
  Apply Name23/1 -> Data Type Conversion9/1

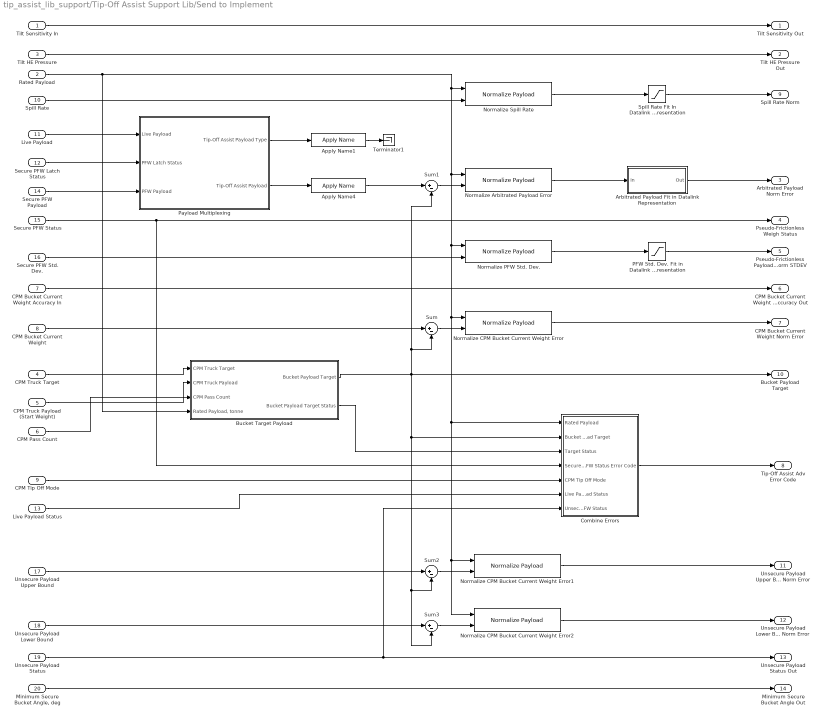
== system tip_assist_lib_support/Tip-Off Assist Support Lib/Send to Implement ==
  Tilt Sensitivity In : Inport
  Rated Payload : Inport  Port=2
  Tilt HE Pressure : Inport  Port=3
  CPM Truck Target : Inport  Port=4
  CPM Truck Payload (Start Weight) : Inport  Port=5
  CPM Pass Count : Inport  Port=6
  CPM Bucket Current Weight Accuracy In : Inport  Port=7
  CPM Bucket Current Weight : Inport  Port=8
  CPM Tip Off Mode : Inport  Port=9
  Spill Rate : Inport  Port=10
  Live Payload : Inport  Port=11
  Secure PFW Latch Status : Inport  Port=12
  Live Payload Status : Inport  Port=13
  Secure PFW Payload : Inport  Port=14
  Secure PFW Status : Inport  Port=15
  Secure PFW Std. Dev. : Inport  Port=16
  Unsecure Payload Upper Bound : Inport  Port=17
  Unsecure Payload Lower Bound : Inport  Port=18
  Unsecure Payload Status : Inport  Port=19
  "Minimum Secure Bucket Angle, deg" : Inport  Port=20
  Apply Name1 : lib_CATutils_Utilities_ApplyName_v2/Apply Name  sigLabel='toa_sendPayloadType'  enTst=true
  Apply Name4 : lib_CATutils_Utilities_ApplyName_v2/Apply Name  sigLabel='toa_sendPayloadArb'  enTst=true
  Arbitrated Payload Fit in Datalink Representation : Subsystem
  Bucket Target Payload : Subsystem
  Combine Errors : Subsystem
  Normalize Arbitrated Payload Error : tip_assist_lib/Normalize Payload
  Normalize CPM Bucket Current Weight Error : tip_assist_lib/Normalize Payload
  Normalize CPM Bucket Current Weight Error1 : tip_assist_lib/Normalize Payload
  Normalize CPM Bucket Current Weight Error2 : tip_assist_lib/Normalize Payload
  Normalize PFW Std. Dev. : tip_assist_lib/Normalize Payload
  Normalize Spill Rate : tip_assist_lib/Normalize Payload
  PFW Std. Dev. Fit in Datalink Representation : Saturate  UpperLimit=175  LowerLimit=0  RndMeth=Nearest
  Payload Multiplexing : Subsystem
  Spill Rate Fit In Datalink Representation : Saturate  UpperLimit=300  LowerLimit=0  RndMeth=Nearest
  Sum{,1..3} (4 alike) : Sum  Inputs=|+-
  Terminator1 : Terminator
  Tilt Sensitivity Out : Outport
  Tilt HE Pressure Out : Outport  Port=2
  Arbitrated Payload Norm Error : Outport  Port=3
  Pseudo-Frictionless Weigh Status : Outport  Port=4
  Pseudo-Frictionless Payload Norm STDEV : Outport  Port=5
  CPM Bucket Current Weight Accuracy Out : Outport  Port=6
  CPM Bucket Current Weight Norm Error : Outport  Port=7
  Tip-Off Assist Adv Error Code : Outport  Port=8
  Spill Rate Norm : Outport  Port=9
  Bucket Payload Target : Outport  Port=10
  Unsecure Payload Upper Bound Norm Error : Outport  Port=11
  Unsecure Payload Lower Bound Norm Error : Outport  Port=12
  Unsecure Payload Status Out : Outport  Port=13
  Minimum Secure Bucket Angle Out : Outport  Port=14
  wires:
  Combine Errors/1(Error Code) -> Tip-Off Assist Adv Error Code/1
  Tilt HE Pressure/1 -> Tilt HE Pressure Out/1
  Secure PFW Status/1 -> Combine Errors/4(Secure PFW Status), Pseudo-Frictionless Weigh Status/1
  Secure PFW Std. Dev./1 -> Normalize PFW Std. Dev./2
  Secure PFW Latch Status/1 -> Payload Multiplexing/2(PFW Latch Status)
  Secure PFW Payload/1 -> Payload Multiplexing/3(PFW Payload)
  Live Payload/1 -> Payload Multiplexing/1(Live Payload)
  Spill Rate/1 -> Normalize Spill Rate/2
  Normalize Spill Rate/1 -> Spill Rate Fit In Datalink Representation/1
  CPM Tip Off Mode/1 -> Combine Errors/5(CPM Tip Off Mode)
  Sum/1 -> Normalize CPM Bucket Current Weight Error/2
  Sum1/1 -> Normalize Arbitrated Payload Error/2
  Normalize Arbitrated Payload Error/1 -> Arbitrated Payload Fit in Datalink Representation/1(In)
  CPM Bucket Current Weight Accuracy In/1 -> CPM Bucket Current Weight Accuracy Out/1
  CPM Bucket Current Weight/1 -> Sum/1
  Payload Multiplexing/1(Tip-Off Assist Payload Type) -> Apply Name1/1
  Payload Multiplexing/2(Tip-Off Assist Payload) -> Apply Name4/1
  Bucket Target Payload/2(Bucket Payload Target Status) -> Combine Errors/3(Target Status)
  Bucket Target Payload/1(Bucket Payload Target) -> Combine Errors/2(Bucket Payload Target), Sum3/2, Sum2/2, Sum/2, Sum1/2, Bucket Payload Target/1
  CPM Truck Target/1 -> Bucket Target Payload/1(CPM Truck Target)
  CPM Truck Payload (Start Weight)/1 -> Bucket Target Payload/2(CPM Truck Payload)
  Tilt Sensitivity In/1 -> Tilt Sensitivity Out/1
  Normalize PFW Std. Dev./1 -> PFW Std. Dev. Fit in Datalink Representation/1
  Normalize CPM Bucket Current Weight Error/1 -> CPM Bucket Current Weight Norm Error/1
  Live Payload Status/1 -> Combine Errors/6(Live Payload Status)
  Rated Payload/1 -> Bucket Target Payload/4("Rated Payload, tonne"), Normalize Arbitrated Payload Error/1, Normalize CPM Bucket Current Weight Error1/1, Normalize CPM Bucket Current Weight Error2/1, Combine Errors/1(Rated Payload), Normalize CPM Bucket Current Weight Error/1, Normalize PFW Std. Dev./1, Normalize Spill Rate/1
  Spill Rate Fit In Datalink Representation/1 -> Spill Rate Norm/1
  PFW Std. Dev. Fit in Datalink Representation/1 -> Pseudo-Frictionless Payload Norm STDEV/1
  Arbitrated Payload Fit in Datalink Representation/1(Out) -> Arbitrated Payload Norm Error/1
  Unsecure Payload Status/1 -> Combine Errors/7(Unsecure PFW Status), Unsecure Payload Status Out/1
  Unsecure Payload Lower Bound/1 -> Sum3/1
  Unsecure Payload Upper Bound/1 -> Sum2/1
  Normalize CPM Bucket Current Weight Error1/1 -> Unsecure Payload Upper Bound Norm Error/1
  Normalize CPM Bucket Current Weight Error2/1 -> Unsecure Payload Lower Bound Norm Error/1
  Sum2/1 -> Normalize CPM Bucket Current Weight Error1/2
  Sum3/1 -> Normalize CPM Bucket Current Weight Error2/2
  "Minimum Secure Bucket Angle, deg"/1 -> Minimum Secure Bucket Angle Out/1
  Apply Name4/1 -> Sum1/1
  Apply Name1/1 -> Terminator1/1
  CPM Pass Count/1 -> Bucket Target Payload/3(CPM Pass Count)

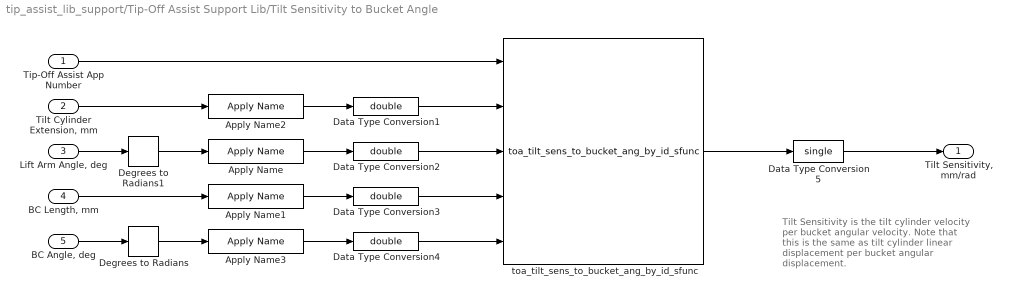
== system tip_assist_lib_support/Tip-Off Assist Support Lib/Tilt Sensitivity to Bucket Angle ==
  note: Tilt Sensitivity is the tilt cylinder velocity per bucket angular velocity.
      | Note that this is the same as tilt cylinder linear displacement per bucket angular displacement.
  Tip-Off Assist App Number : Inport
  "Tilt Cylinder Extension, mm" : Inport  Port=2
  "Lift Arm Angle, deg" : Inport  Port=3
  "BC Length, mm" : Inport  Port=4
  "BC Angle, deg" : Inport  Port=5
  Apply Name : lib_CATutils_Utilities_ApplyName_v2/Apply Name  sigLabel='toa_inTsLiftAngle'  enTst=true
  Apply Name1 : lib_CATutils_Utilities_ApplyName_v2/Apply Name  sigLabel='toa_inTsBc'  enTst=true
  Apply Name2 : lib_CATutils_Utilities_ApplyName_v2/Apply Name  sigLabel='toa_inTsTiltExt'  enTst=true
  Apply Name3 : lib_CATutils_Utilities_ApplyName_v2/Apply Name  sigLabel='toa_inTsBcAng'  enTst=true
  Data Type Conversion{1..4} (4 alike) : DataTypeConversion  OutDataTypeStr=double  SaturateOnIntegerOverflow=on  RndMeth=Zero
      settings: AttributesFormatString=Output Data Type: %<OutDataTypeStr>\n
  Data Type Conversion5 : DataTypeConversion  OutDataTypeStr=single  SaturateOnIntegerOverflow=on  RndMeth=Zero
      settings: AttributesFormatString=Output Data Type: %<OutDataTypeStr>\n
  Degrees to Radians : simulink_extras/Transformations/Degrees to Radians
  Degrees to Radians1 : simulink_extras/Transformations/Degrees to Radians
  toa_tilt_sens_to_bucket_ang_by_id_sfunc : S-Function  FunctionName=toa_tilt_sens_to_bucket_ang_by_id_sfunc  SFunctionDeploymentMode=off  EnableBusSupport=off  mask(Legacy Function){SFunctionSpec=void toa_tilt_sens_to_bucket_ang_by_id(uint32 u1, double u2, double u3, double u4, double u5, double y1[1]), ShowSpec=on}
      mask prompts: ShowSpec "Display function specification"
      mask help:
      | This block allows you to call the legacy functions specified by the following Legacy Code Tool definition:
      | def.SFunctionName = 'toa_tilt_sens_to_bucket_ang_by_id_sfunc';
      | def.OutputFcnSpec = 'void toa_tilt_sens_to_bucket_ang_by_id(uint32 u1, double u2, double u3, double u4, double u5, double y1[1])';
      | def.HeaderFiles = {'tipoff_assist.h'};
      | def.SourceFiles = {'tipoff_assist.c'};
      | def.IncPaths = {'./c_src'};
      mask Help: <p>This block was generated automatically by the Legacy Code Tool. For detailed help on this tool, call<a href="matlab:legacy_code('help')"> legacy_code('help')</a>.</p>
      mask Callback ShowSpec:
      | if strcmp(get_param(gcbh, 'ShowSpec'), 'on')
      |   set_param(gcbh, 'MaskDisplay', sprintf('fprintf(''%s'');', get_param(gcbh, 'SFunctionSpec')));
      | else
      |   set_param(gcbh, 'MaskDisplay', sprintf('fprintf(''%s'');', get_param(gcbh, 'FunctionName')));
      | end
      mask Display: fprintf('%s','void toa_tilt_sens_to_bucket_ang_by_id(uint32 u1, double u2, double u3, double u4, double u5, double y1[1])');
  "Tilt Sensitivity, mm/rad" : Outport
  wires:
  Degrees to Radians/1 -> Apply Name3/1
  "BC Angle, deg"/1 -> Degrees to Radians/1
  Degrees to Radians1/1 -> Apply Name/1
  "Lift Arm Angle, deg"/1 -> Degrees to Radians1/1
  Apply Name3/1 -> Data Type Conversion4/1
  Apply Name/1 -> Data Type Conversion2/1
  Apply Name2/1 -> Data Type Conversion1/1
  Apply Name1/1 -> Data Type Conversion3/1
  Data Type Conversion5/1 -> "Tilt Sensitivity, mm/rad"/1
  Data Type Conversion4/1 -> toa_tilt_sens_to_bucket_ang_by_id_sfunc/5
  Data Type Conversion3/1 -> toa_tilt_sens_to_bucket_ang_by_id_sfunc/4
  Data Type Conversion1/1 -> toa_tilt_sens_to_bucket_ang_by_id_sfunc/2
  Data Type Conversion2/1 -> toa_tilt_sens_to_bucket_ang_by_id_sfunc/3
  "BC Length, mm"/1 -> Apply Name1/1
  toa_tilt_sens_to_bucket_ang_by_id_sfunc/1 -> Data Type Conversion5/1
  "Tilt Cylinder Extension, mm"/1 -> Apply Name2/1
  Tip-Off Assist App Number/1 -> toa_tilt_sens_to_bucket_ang_by_id_sfunc/1
